simulink model "v7_2025_11_28_D2_work_in_progress"  (R2025a)
settings: Solver=FixedStepAuto  StartTime=0.0  StopTime=120  FixedStep=1e-3  RelTol=1e-3  EnableMultiTasking=on
undefined symbols (not defined in the file): A0, A1, D0, D1, D10, D11, D12, D13, D2, D3, D4, D5, D6, D7, D8, D9, PTA0, PTA1, PTA2, PTB2, PTB23, PTB3, PTB9, PTC16, PTC17, PTC2, PTC3, PTC4, PTD0, PTD1, PTD2, PTD3
libraries: frdmk64flib x19, etargetslib x2, dspstat3 x1
settings Model: ExtModeTrigDuration=5  Creator=School Account  LastModifiedBy=School Account
settings SolverCC: AlgebraicLoopSolver=TrustRegion  AutoInsertRateTranBlk=on
settings OptimizationCC: DefaultParameterBehavior=Inlined  EnhancedBackFolding=on  PassReuseOutputArgsAs=Individual arguments  ZeroExternalMemoryAtStartup=off  ZeroInternalMemoryAtStartup=off  MaxStackSize=64  OptimizeBlockOrder=speed  DifferentSizesBufferReuse=on  OptimizationCustomize=off  EfficientTunableParamExpr=on
settings DebuggingCC: ParameterTunabilityLossMsg=error
settings HardwareCC: ProdBitPerPointer=32.0  ProdBitPerSizeT=32.0  ProdBitPerPtrDiffT=32.0  ProdLargestAtomicInteger=Long  ProdLargestAtomicFloat=Double  ProdWordSize=32.0  ProdHWDeviceType=ARM Compatible->ARM Cortex
settings SFSimCC: MATLABDynamicMemAlloc=off
settings RTWCC: SystemTargetFile=ert.tlc  HardwareBoard=NXP FRDM-K64F  TLCOptions="-aInlineSetEventsForThisBaseRateFcn=TLC_FALSE -aSuppressMultiTaskScheduler=TLC_FALSE  -aRateBasedStepFcn=0"  TemplateMakefile=ert_default_tmf  Toolchain=GNU Tools for ARM Embedded Processors  GPUComputeCapability=3.5  Description=Embedded Coder
settings CodeAppCC: ForceParamTrailComments=on  IgnoreCustomStorageClasses=off  OperatorAnnotations=on  SimulinkDataObjDesc=on  SFDataObjDesc=on  InsertBlockDesc=on
settings ERTTargetCC: ExtModeTransport=4.0  ExtModeStaticAlloc=off  ExtModeMexFile=sendToCommService  ExtModeIntrfLevel=Level1  DynamicArrayContainerType=coder::array

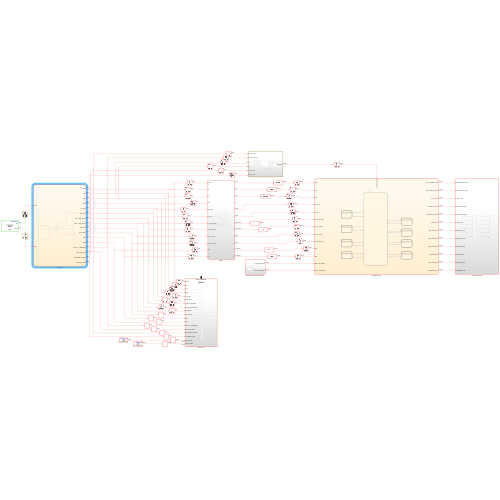
[thumbnail: Simulink's stored preview of the top-level diagram]
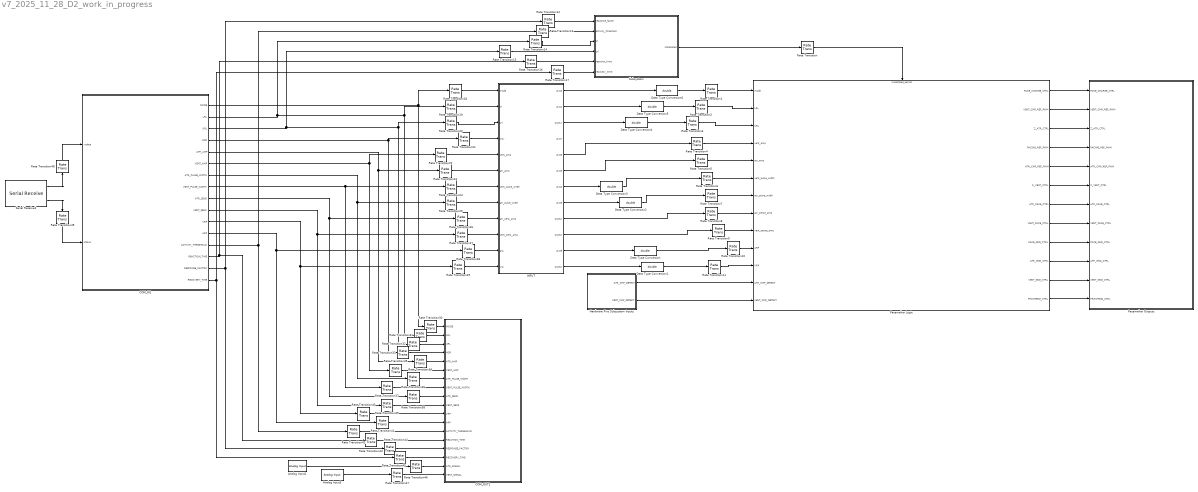
== system v7_2025_11_28_D2_work_in_progress ==
  Analog Input2 : frdmk64flib/Analog Input  Whichpin=PTB2 (A0)  SampleTime=-1
  Analog Input3 : frdmk64flib/Analog Input  Whichpin=PTB3 (A1)  SampleTime=-1
  COM_IN1 : Stateflow chart  TreatAsAtomicUnit=on
  COM_OUT1 : Subsystem  TreatAsAtomicUnit=on
  Data Type Conversion{,1..6} (7 alike) : DataTypeConversion  OutDataTypeStr=double  SaturateOnIntegerOverflow=off  RndMeth=Floor
  Hardware Pins Subsystem Inputs : Subsystem
  "INPUT " : Subsystem
  Pacemaker Logic : Stateflow chart  TreatAsAtomicUnit=on
      settings: PortSchema="{\"entries\":[{\"content\":{\"sides\":[{\"content\":{\"connectorIds\":[\"In1\",\"In4\",\"In13\",\"In5\",\"In2\",\"In6\",\"In3\",\"In7\",\"In10\",\"In8\",\"In11\",\"In9\",\"In12\"]},\"type\":\"ConnectorPlacement.EquallySpacedRectSide\",\"uuid\":\"2821f65a-9b3e-4ca7-babd-b0602bfdca31\"},{\"content\":{\"connectorIds\":[\"Out1\",\"Out2\",\"Out3\",\"Out4\",\"Out5\",\"Out6\",\"Out7\",\"Out8\",\"Out9\",\"Out10\",\"Out11\",\"Out12\"],\"side\":\"RIGHT\"},\"type\":\"ConnectorPlacement.EquallySpacedRectSide\",\"uuid\":\"3302ad84-7e85-4bae-9388-240b69681e7f\"},{\"content\":{\"connectorIds\":[\"In14\"],\"side\":\"TOP\"},\"type\":\"ConnectorPlacement.EquallySpacedRectSide\",\"uuid\":\"cc666da6-1c79-42dc-9f95-9791247ae8bf\"},{\"content\":{\"side\":\"BOTTOM\"},\"type\":\"ConnectorPlacement.EquallySpacedRectSide\",\"uuid\":\"6c7eefe5-bab4-42c2-8766-4f3cee9532f0\"}]},\"type\":\"ConnectorPlacement.EquallySpacedConnector\",\"uuid\":\"e2a43bfa-d126-4f35-adbf-2cf33da0501f\"}],\"packageUris\":[\"http://schema.mathworks.com/mf0/Connector/R2020b\"],\"version\":\"1.0\"}"
  Pacemaker Outputs : Subsystem
  Rate Transition{,1..49} (50 alike) : RateTransition  OutPortSampleTime=0.001
  Serial Receive2 : frdmk64flib/Serial Receive  SCIModule=0  Baudrate=uint32(9600)  Parity=None  StopBits=1  HardwareFlowControl=None  ByteOrder=LittleEndian  DataType=uint8  DataLength=18  BlockingMode=off  OutputStatus=on  SampleTime=0.01
  Subsystem : Subsystem
  wires:
  Pacemaker Logic/1(PACE_CHARGE_CTRL) -> Pacemaker Outputs/1(PACE_CHARGE_CTRL)
  Pacemaker Logic/3(Z_ATR_CTRL) -> Pacemaker Outputs/3(Z_ATR_CTRL)
  Pacemaker Logic/4(PACING_REF_PWM) -> Pacemaker Outputs/4(PACING_REF_PWM)
  Pacemaker Logic/7(ATR_PACE_CTRL) -> Pacemaker Outputs/7(ATR_PACE_CTRL)
  Pacemaker Logic/9(PACE_GND_CTRL) -> Pacemaker Outputs/9(PACE_GND_CTRL)
  Pacemaker Logic/10(ATR_GND_CTRL) -> Pacemaker Outputs/10(ATR_GND_CTRL)
  Pacemaker Logic/11(VENT_GND_CTRL) -> Pacemaker Outputs/11(VENT_GND_CTRL)
  Pacemaker Logic/8(VENT_PACE_CTRL) -> Pacemaker Outputs/8(VENT_PACE_CTRL)
  Pacemaker Logic/6(Z_VENT_CTRL) -> Pacemaker Outputs/6(Z_VENT_CTRL)
  Pacemaker Logic/12(FRONTEND_CTRL) -> Pacemaker Outputs/12(FRONTEND_CTRL)
  Pacemaker Logic/5(ATR_CMP_REF_PWM) -> Pacemaker Outputs/5(ATR_CMP_REF_PWM)
  Pacemaker Logic/2(VENT_CMP_REF_PWM) -> Pacemaker Outputs/2(VENT_CMP_REF_PWM)
  Hardware Pins Subsystem Inputs/2(VENT_CMP_DETECT) -> Pacemaker Logic/12(VENT_CMP_DETECT)
  Hardware Pins Subsystem Inputs/1(ATR_CMP_DETECT) -> Pacemaker Logic/9(ATR_CMP_DETECT)
  "INPUT "/11(Out9) -> Data Type Conversion/1
  "INPUT "/12(Out10) -> Data Type Conversion1/1
  "INPUT "/10(Out13) -> Rate Transition9/1
  "INPUT "/9(Out12) -> Rate Transition8/1
  "INPUT "/8(Out5) -> Data Type Conversion2/1
  "INPUT "/7(Out4) -> Data Type Conversion3/1
  "INPUT "/6(Out3) -> Rate Transition5/1
  "INPUT "/5(Out6) -> Rate Transition4/1
  "INPUT "/1(Out2) -> Data Type Conversion6/1
  "INPUT "/2(Out1) -> Data Type Conversion5/1
  "INPUT "/3(Out11) -> Data Type Conversion4/1
  Subsystem/1(Modulated) -> Rate Transition/1
  Analog Input3/1 -> Rate Transition47/1
  Analog Input2/1 -> Rate Transition46/1
  Serial Receive2/1 -> Rate Transition48/1
  Serial Receive2/2 -> Rate Transition49/1
  COM_IN1/1(MODE) -> Rate Transition18/1, Rate Transition30/1
  COM_IN1/2(LRL) -> Rate Transition14/1, Rate Transition31/1, Rate Transition19/1
  COM_IN1/3(URL) -> Rate Transition15/1, Rate Transition32/1, Rate Transition20/1
  COM_IN1/4(MSR) -> Rate Transition21/1, Rate Transition33/1
  COM_IN1/5(ATR_AMP) -> Rate Transition34/1, Rate Transition23/1
  COM_IN1/6(VENT_AMP) -> Rate Transition22/1, Rate Transition35/1
  COM_IN1/7(ATR_PULSE_WIDTH) -> Rate Transition36/1, Rate Transition25/1
  COM_IN1/8(VENT_PULSE_WIDTH) -> Rate Transition37/1, Rate Transition24/1
  COM_IN1/9(ATR_SENS) -> Rate Transition26/1, Rate Transition38/1
  COM_IN1/10(VENT_SENS) -> Rate Transition27/1, Rate Transition39/1
  COM_IN1/11(VRP) -> Rate Transition29/1, Rate Transition40/1
  COM_IN1/12(ARP) -> Rate Transition28/1, Rate Transition41/1
  COM_IN1/13(ACTIVITY_THRESHOLD) -> Rate Transition13/1, Rate Transition42/1
  COM_IN1/14(REACTION_TIME) -> Rate Transition16/1, Rate Transition43/1
  COM_IN1/15(RESPONSE_FACTOR) -> Rate Transition12/1, Rate Transition44/1
  COM_IN1/16(RECOVERY_TIME) -> Rate Transition17/1, Rate Transition45/1
  Rate Transition/1 -> Pacemaker Logic/14(modulated_period)
  Rate Transition1/1 -> Pacemaker Logic/1(mode)
  Rate Transition2/1 -> Pacemaker Logic/4(LRL)
  Rate Transition3/1 -> Pacemaker Logic/13(URL)
  Rate Transition4/1 -> Pacemaker Logic/5(vent_amp)
  Rate Transition5/1 -> Pacemaker Logic/2(atr_amp)
  Rate Transition6/1 -> Pacemaker Logic/6(vent_pulse_width)
  Rate Transition7/1 -> Pacemaker Logic/3(atr_pulse_width)
  Rate Transition8/1 -> Pacemaker Logic/7(atr_sense_amp)
  Rate Transition9/1 -> Pacemaker Logic/10(vent_sense_amp)
  Rate Transition10/1 -> Pacemaker Logic/8(ARP)
  Rate Transition11/1 -> Pacemaker Logic/11(VRP)
  Rate Transition12/1 -> Subsystem/1(response_factor)
  Rate Transition13/1 -> Subsystem/2(activity_threshold)
  Rate Transition14/1 -> Subsystem/3(lrl)
  Rate Transition15/1 -> Subsystem/4(url)
  Rate Transition16/1 -> Subsystem/5(reaction_time)
  Rate Transition17/1 -> Subsystem/6(recovery_time)
  Rate Transition18/1 -> "INPUT "/1(mode)
  Rate Transition19/1 -> "INPUT "/2(lrl)
  Rate Transition20/1 -> "INPUT "/3(url)
  Rate Transition21/1 -> "INPUT "/4(msr)
  Rate Transition22/1 -> "INPUT "/5(vent_amp)
  Rate Transition23/1 -> "INPUT "/6(atr_amp)
  Rate Transition24/1 -> "INPUT "/7(vent_pulse_width)
  Rate Transition25/1 -> "INPUT "/8(atr_pulse_width)
  Rate Transition26/1 -> "INPUT "/9(atr_sens_amp)
  Rate Transition27/1 -> "INPUT "/10(vent_sens_amp)
  Rate Transition28/1 -> "INPUT "/11(arp)
  Rate Transition29/1 -> "INPUT "/12(vrp)
  Rate Transition30/1 -> COM_OUT1/1(MODE)
  Rate Transition31/1 -> COM_OUT1/2(LRL)
  Rate Transition32/1 -> COM_OUT1/3(URL)
  Rate Transition33/1 -> COM_OUT1/4(MSR)
  Rate Transition34/1 -> COM_OUT1/5(ATR_AMP)
  Rate Transition35/1 -> COM_OUT1/6(VENT_AMP)
  Rate Transition36/1 -> COM_OUT1/7(ATR_PULSE_WIDTH)
  Rate Transition37/1 -> COM_OUT1/8(VENT_PULSE_WIDTH)
  Rate Transition38/1 -> COM_OUT1/9(ATR_SENS)
  Rate Transition39/1 -> COM_OUT1/10(VENT_SENS)
  Rate Transition40/1 -> COM_OUT1/11(VRP)
  Rate Transition41/1 -> COM_OUT1/12(ARP)
  Rate Transition42/1 -> COM_OUT1/13(ACTIVITY_THRESHOLD)
  Rate Transition43/1 -> COM_OUT1/14(REACTION_TIME)
  Rate Transition44/1 -> COM_OUT1/15(RESPONSE_FACTOR)
  Rate Transition45/1 -> COM_OUT1/16(RECOVERY_TIME)
  Rate Transition46/1 -> COM_OUT1/17(ATR_SIGNAL)
  Rate Transition47/1 -> COM_OUT1/18(VENT_SIGNAL)
  Rate Transition48/1 -> COM_IN1/1(rxdata)
  Rate Transition49/1 -> COM_IN1/2(status)
  Data Type Conversion/1 -> Rate Transition10/1
  Data Type Conversion1/1 -> Rate Transition11/1
  Data Type Conversion2/1 -> Rate Transition7/1
  Data Type Conversion3/1 -> Rate Transition6/1
  Data Type Conversion4/1 -> Rate Transition3/1
  Data Type Conversion5/1 -> Rate Transition2/1
  Data Type Conversion6/1 -> Rate Transition1/1

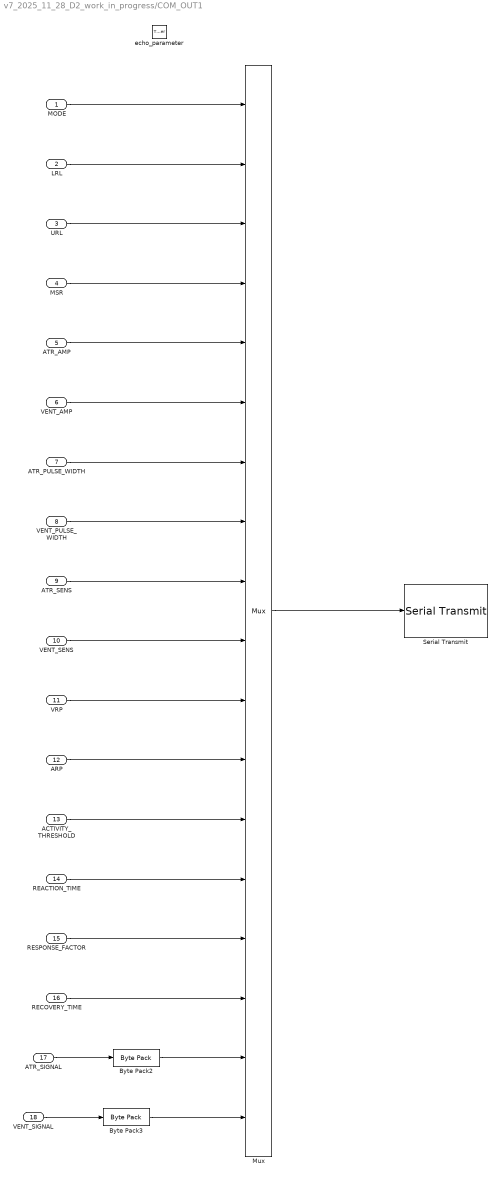
== system v7_2025_11_28_D2_work_in_progress/COM_OUT1 ==
  MODE : Inport
  LRL : Inport  Port=2
  URL : Inport  Port=3
  MSR : Inport  Port=4
  ATR_AMP : Inport  Port=5
  VENT_AMP : Inport  Port=6
  ATR_PULSE_WIDTH : Inport  Port=7
  VENT_PULSE_WIDTH : Inport  Port=8
  ATR_SENS : Inport  Port=9
  VENT_SENS : Inport  Port=10
  VRP : Inport  Port=11
  ARP : Inport  Port=12
  ACTIVITY_THRESHOLD : Inport  Port=13
  REACTION_TIME : Inport  Port=14
  RESPONSE_FACTOR : Inport  Port=15
  RECOVERY_TIME : Inport  Port=16
  ATR_SIGNAL : Inport  Port=17  OutDataTypeStr=double
  VENT_SIGNAL : Inport  Port=18  OutDataTypeStr=double
  echo_parameter : TriggerPort  TriggerType=function-call  IsSimulinkFunction=on  FunctionName=echo_parameter  VariantControl=(inherit)
  Byte Pack2 : etargetslib/Byte Pack  datatypes={'double'}  byteAlign=1
  Byte Pack3 : etargetslib/Byte Pack  datatypes={'double'}  byteAlign=1
  Mux : Mux  Inputs=18
  Serial Transmit : frdmk64flib/Serial Transmit  SCIModule=0  Baudrate=uint32(9600)  Parity=None  StopBits=1  HardwareFlowControl=None  ByteOrder=LittleEndian  BlockingMode=on  OutputStatus=off
  wires:
  VENT_SIGNAL/1 -> Byte Pack3/1
  ATR_SIGNAL/1 -> Byte Pack2/1
  Byte Pack2/1 -> Mux/17
  Byte Pack3/1 -> Mux/18
  Mux/1 -> Serial Transmit/1
  MODE/1 -> Mux/1
  LRL/1 -> Mux/2
  URL/1 -> Mux/3
  MSR/1 -> Mux/4
  ATR_AMP/1 -> Mux/5
  VENT_AMP/1 -> Mux/6
  ATR_PULSE_WIDTH/1 -> Mux/7
  VENT_PULSE_WIDTH/1 -> Mux/8
  ATR_SENS/1 -> Mux/9
  VENT_SENS/1 -> Mux/10
  VRP/1 -> Mux/11
  ARP/1 -> Mux/12
  ACTIVITY_THRESHOLD/1 -> Mux/13
  REACTION_TIME/1 -> Mux/14
  RESPONSE_FACTOR/1 -> Mux/15
  RECOVERY_TIME/1 -> Mux/16

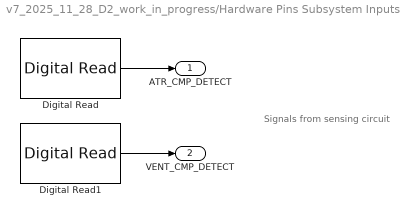
== system v7_2025_11_28_D2_work_in_progress/Hardware Pins Subsystem Inputs ==
  note: Signals from sensing circuit
  Digital Read : frdmk64flib/Digital Read  Whichpin=PTC16 (D0)  SampleTime=-1
  Digital Read1 : frdmk64flib/Digital Read  Whichpin=PTC17 (D1)  SampleTime=-1
  ATR_CMP_DETECT : Outport
  VENT_CMP_DETECT : Outport  Port=2
  wires:
  Digital Read1/1 -> VENT_CMP_DETECT/1
  Digital Read/1 -> ATR_CMP_DETECT/1

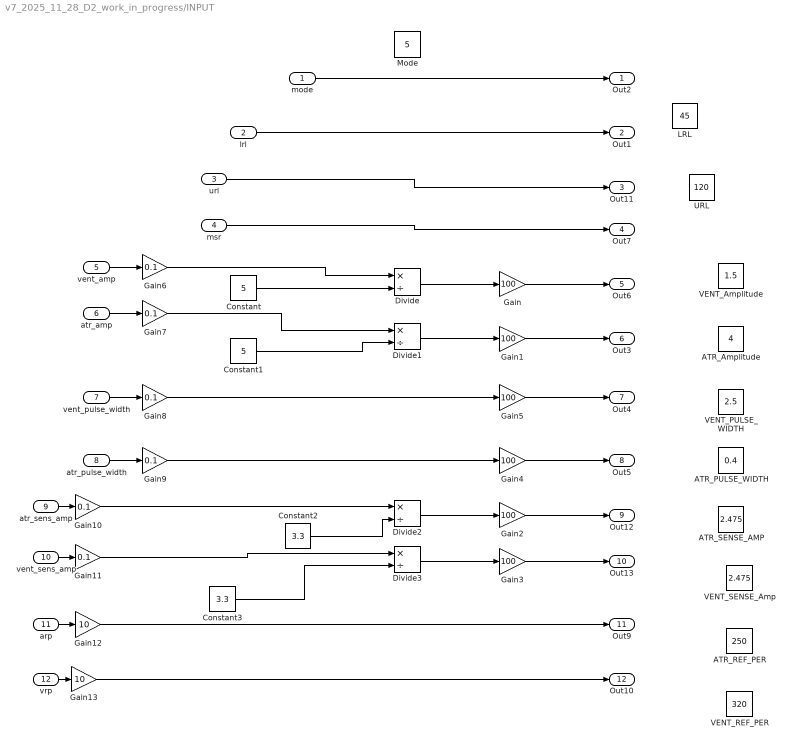
== system v7_2025_11_28_D2_work_in_progress/INPUT  ==
  mode : Inport
  lrl : Inport  Port=2
  url : Inport  Port=3
  msr : Inport  Port=4
  vent_amp : Inport  Port=5
  atr_amp : Inport  Port=6
  vent_pulse_width : Inport  Port=7
  atr_pulse_width : Inport  Port=8
  atr_sens_amp : Inport  Port=9
  vent_sens_amp : Inport  Port=10
  arp : Inport  Port=11
  vrp : Inport  Port=12
  ATR_Amplitude : Constant  Value=4
  ATR_PULSE_WIDTH : Constant  Value=0.4
  ATR_REF_PER : Constant  Value=250
  ATR_SENSE_AMP : Constant  Value=2.475
  Constant : Constant  Value=5
  Constant1 : Constant  Value=5
  Constant2 : Constant  Value=3.3
  Constant3 : Constant  Value=3.3
  Divide{,1..3} (4 alike) : Product  Inputs=*/
  Gain{,1..5} (6 alike) : Gain  Gain=100
  Gain{6..11} (6 alike) : Gain  Gain=0.1
  Gain12 : Gain  Gain=10
  Gain13 : Gain  Gain=10
  LRL : Constant  Value=45
  Mode : Constant  Value=5
  URL : Constant  Value=120
  VENT_Amplitude : Constant  Value=1.5
  VENT_PULSE_WIDTH : Constant  Value=2.5
  VENT_REF_PER : Constant  Value=320
  VENT_SENSE_Amp : Constant  Value=2.475
  Out2 : Outport
  Out1 : Outport  Port=2
  Out11 : Outport  Port=3
  Out7 : Outport  Port=4
  Out6 : Outport  Port=5
  Out3 : Outport  Port=6
  Out4 : Outport  Port=7
  Out5 : Outport  Port=8
  Out12 : Outport  Port=9
  Out13 : Outport  Port=10
  Out9 : Outport  Port=11
  Out10 : Outport  Port=12
  wires:
  Gain/1 -> Out6/1
  Gain1/1 -> Out3/1
  Gain2/1 -> Out12/1
  Gain3/1 -> Out13/1
  Gain5/1 -> Out4/1
  Gain4/1 -> Out5/1
  Divide/1 -> Gain/1
  Constant/1 -> Divide/2
  Divide1/1 -> Gain1/1
  Constant1/1 -> Divide1/2
  Divide2/1 -> Gain2/1
  Constant2/1 -> Divide2/2
  Divide3/1 -> Gain3/1
  Constant3/1 -> Divide3/2
  vent_amp/1 -> Gain6/1
  mode/1 -> Out2/1
  lrl/1 -> Out1/1
  url/1 -> Out11/1
  msr/1 -> Out7/1
  atr_amp/1 -> Gain7/1
  vent_pulse_width/1 -> Gain8/1
  Gain8/1 -> Gain5/1
  atr_pulse_width/1 -> Gain9/1
  Gain9/1 -> Gain4/1
  atr_sens_amp/1 -> Gain10/1
  Gain6/1 -> Divide/1
  Gain7/1 -> Divide1/1
  Gain10/1 -> Divide2/1
  vent_sens_amp/1 -> Gain11/1
  Gain11/1 -> Divide3/1
  arp/1 -> Gain12/1
  vrp/1 -> Gain13/1
  Gain12/1 -> Out9/1
  Gain13/1 -> Out10/1

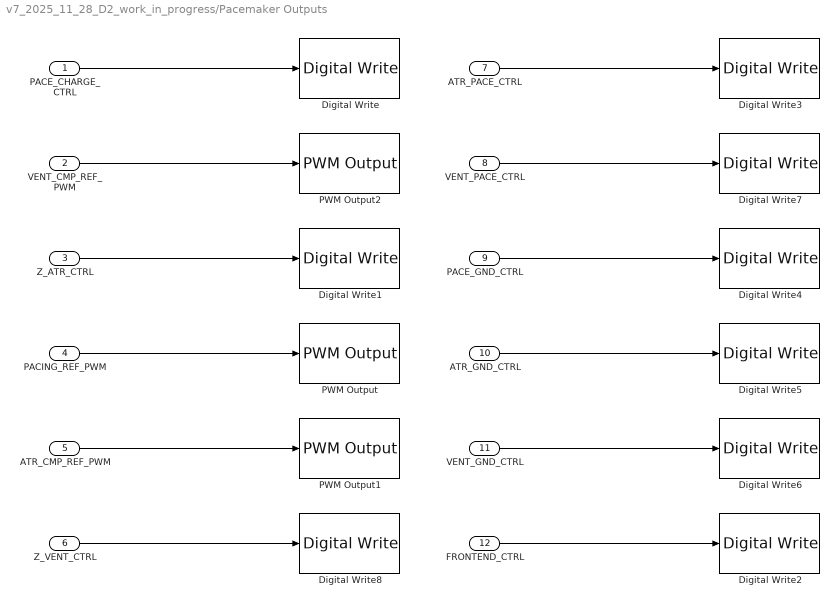
== system v7_2025_11_28_D2_work_in_progress/Pacemaker Outputs ==
  PACE_CHARGE_CTRL : Inport
  VENT_CMP_REF_PWM : Inport  Port=2
  Z_ATR_CTRL : Inport  Port=3
  PACING_REF_PWM : Inport  Port=4
  ATR_CMP_REF_PWM : Inport  Port=5
  Z_VENT_CTRL : Inport  Port=6
  ATR_PACE_CTRL : Inport  Port=7
  VENT_PACE_CTRL : Inport  Port=8
  PACE_GND_CTRL : Inport  Port=9
  ATR_GND_CTRL : Inport  Port=10
  VENT_GND_CTRL : Inport  Port=11
  FRONTEND_CTRL : Inport  Port=12
  Digital Write : frdmk64flib/Digital Write  Whichpin=PTB9 (D2)
  Digital Write1 : frdmk64flib/Digital Write  Whichpin=PTB23 (D4)
  Digital Write2 : frdmk64flib/Digital Write  Whichpin=PTD1 (D13)
  Digital Write3 : frdmk64flib/Digital Write  Whichpin=PTA0 (D8)
  Digital Write4 : frdmk64flib/Digital Write  Whichpin=PTD0 (D10)
  Digital Write5 : frdmk64flib/Digital Write  Whichpin=PTD2 (D11)
  Digital Write6 : frdmk64flib/Digital Write  Whichpin=PTD3 (D12)
  Digital Write7 : frdmk64flib/Digital Write  Whichpin=PTC4 (D9)
  Digital Write8 : frdmk64flib/Digital Write  Whichpin=PTC3 (D7)
  PWM Output : frdmk64flib/PWM Output  Whichpin=PTA2 (D5)  InitialFrequency=2000  InitialDutyCycle=0
  PWM Output1 : frdmk64flib/PWM Output  Whichpin=PTC2 (D6)  InitialFrequency=2000  InitialDutyCycle=0
  PWM Output2 : frdmk64flib/PWM Output  Whichpin=PTA1 (D3)  InitialFrequency=2000  InitialDutyCycle=0
  wires:
  PACE_CHARGE_CTRL/1 -> Digital Write/1
  Z_ATR_CTRL/1 -> Digital Write1/1
  PACING_REF_PWM/1 -> PWM Output/1
  ATR_PACE_CTRL/1 -> Digital Write3/1
  PACE_GND_CTRL/1 -> Digital Write4/1
  ATR_GND_CTRL/1 -> Digital Write5/1
  VENT_GND_CTRL/1 -> Digital Write6/1
  VENT_PACE_CTRL/1 -> Digital Write7/1
  Z_VENT_CTRL/1 -> Digital Write8/1
  FRONTEND_CTRL/1 -> Digital Write2/1
  ATR_CMP_REF_PWM/1 -> PWM Output1/1
  VENT_CMP_REF_PWM/1 -> PWM Output2/1

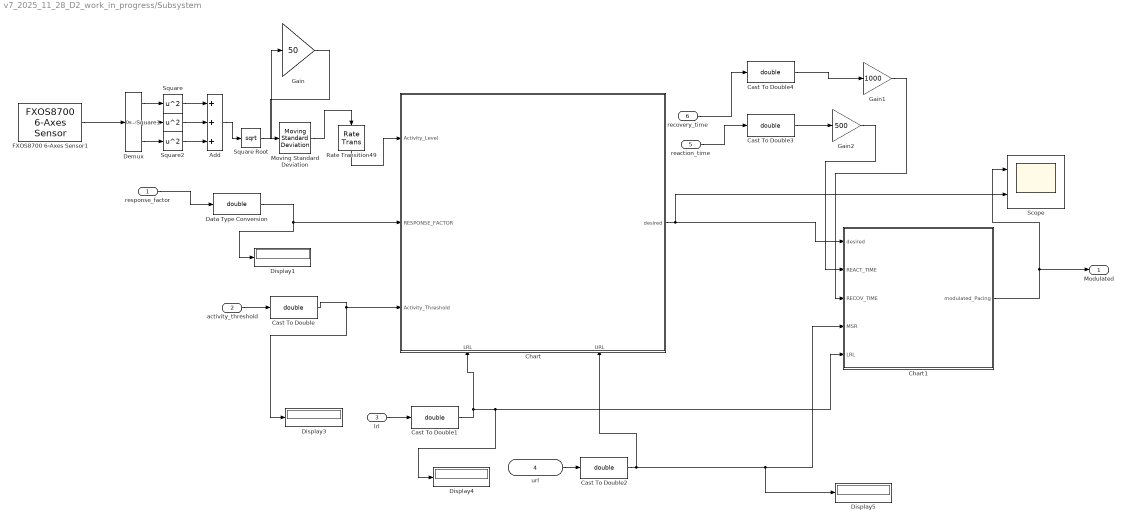
== system v7_2025_11_28_D2_work_in_progress/Subsystem ==
  response_factor : Inport
  activity_threshold : Inport  Port=2
  lrl : Inport  Port=3
  url : Inport  Port=4
  reaction_time : Inport  Port=5
  recovery_time : Inport  Port=6
  Add : Sum  Inputs=+++
  Cast To Double{,1..4} (5 alike) : DataTypeConversion  OutDataTypeStr=double  SaturateOnIntegerOverflow=off  RndMeth=Floor
  Chart : Stateflow chart  TreatAsAtomicUnit=on
      settings: PortSchema="{\"entries\":[{\"content\":{\"sides\":[{\"content\":{\"connectorIds\":[\"In3\",\"In4\",\"In5\"]},\"type\":\"ConnectorPlacement.EquallySpacedRectSide\",\"uuid\":\"74c786d3-d2a6-437e-8bb7-c9d9b4a74617\"},{\"content\":{\"connectorIds\":[\"Out1\"],\"side\":\"RIGHT\"},\"type\":\"ConnectorPlacement.EquallySpacedRectSide\",\"uuid\":\"2c46704d-1ce5-4a26-9635-57e0f6503ead\"},{\"content\":{\"side\":\"TOP\"},\"type\":\"ConnectorPlacement.EquallySpacedRectSide\",\"uuid\":\"1e7c0bb1-a8b6-49e0-9e63-e8e48adc5546\"},{\"content\":{\"connectorIds\":[\"In1\",\"In2\"],\"side\":\"BOTTOM\"},\"type\":\"ConnectorPlacement.EquallySpacedRectSide\",\"uuid\":\"98fe2a4d-8dd5-42bc-97d4-b5234350e537\"}]},\"type\":\"ConnectorPlacement.EquallySpacedConnector\",\"uuid\":\"114a6ead-843c-4291-bcbc-4dc58f15d580\"}],\"packageUris\":[\"http://schema.mathworks.com/mf0/Connector/R2020b\"],\"version\":\"1.0\"}"
  Chart1 : Stateflow chart  TreatAsAtomicUnit=on
  Data Type Conversion : DataTypeConversion  OutDataTypeStr=double  SaturateOnIntegerOverflow=off  RndMeth=Floor
  Demux : Demux  Outputs=3
  Display{1,3..5} (4 alike) : Display
  FXOS8700 6-Axes Sensor1 : frdmk64flib/FXOS8700 6-Axes Sensor  Activesensor=Accelerometer only  ODR=800Hz  HybridODR=400Hz  Accelfullrange=-4g to +4g  SampleTime=0.01
  Gain : Gain  Gain=50
  Gain1 : Gain  Gain=1000
  Gain2 : Gain  Gain=500
  Moving Standard Deviation : dspstat3/Moving Standard Deviation  Method=Sliding window  ForgettingFactorPort=off  SpecifyWindowLength=on  WindowLength=128  OverlapLength=127  AllowArbitraryInputLength=off  ForgettingFactor=0.9  SimulateUsing=Interpreted execution
  Rate Transition49 : RateTransition  OutPortSampleTime=0.001
  Scope : Scope  NumInputPorts=2
      settings: ActiveDisplayYMinimum=34.87115106781259  ActiveDisplayYMaximum=115.78130537109008
  Square : Math  Operator=square
  Square Root : Sqrt
  Square1 : Math  Operator=square
  Square2 : Math  Operator=square
  Modulated : Outport
  wires:
  Square1/1 -> Add/2
  Demux/1 -> Square/1
  Square2/1 -> Add/3
  Square/1 -> Add/1
  Demux/2 -> Square1/1
  Demux/3 -> Square2/1
  Add/1 -> Square Root/1
  FXOS8700 6-Axes Sensor1/1 -> Demux/1
  Chart1/1(modulated_Pacing) -> Modulated/1, Scope/1
  Chart/1(desired) -> Chart1/1(desired), Scope/2
  Square Root/1 -> Gain/1
  Gain/1 -> Moving Standard Deviation/1
  response_factor/1 -> Data Type Conversion/1
  Data Type Conversion/1 -> Display1/1, Chart/4(RESPONSE_FACTOR)
  activity_threshold/1 -> Cast To Double/1
  lrl/1 -> Cast To Double1/1
  url/1 -> Cast To Double2/1
  Cast To Double1/1 -> Display4/1, Chart1/5(LRL), Chart/1(LRL)
  Cast To Double2/1 -> Chart/2(URL), Display5/1, Chart1/4(MSR)
  recovery_time/1 -> Cast To Double4/1
  reaction_time/1 -> Cast To Double3/1
  Cast To Double4/1 -> Gain1/1
  Cast To Double/1 -> Chart/5(Activity_Threshold), Display3/1
  Gain1/1 -> Chart1/3(RECOV_TIME)
  Cast To Double3/1 -> Gain2/1
  Gain2/1 -> Chart1/2(REACT_TIME)
  Moving Standard Deviation/1 -> Rate Transition49/1
  Rate Transition49/1 -> Chart/3(Activity_Level)

== stateflow chart v7_2025_11_28_D2_work_in_progress/Subsystem/Chart ==
  state UpperLimiter [commented out]
    entry:
    desired = URL
  state LinearFunction
    during:
    desired = RESPONSE_FACTOR * (Activity_Level  -  Activity_Threshold) + LRL
    % 2. Apply Upper Limit (Clamp to URL)
    if desired > URL
    desired = URL;
    % 3. Apply Lower Limit (Clamp to LRL)
    elseif desired < LRL
    desired = LRL;
    end
  state Init
    entry:
    desired = LRL
  state Start
  state LowerLimiter [commented out]
    entry:
    desired = LRL
  LinearFunction -> UpperLimiter [commented out] : [desired > URL]
  UpperLimiter -> LinearFunction [commented out] : [desired <= URL]
  (default) -> Init
  Init -> Start
  Start -> LinearFunction : [Activity_Level >= Activity_Threshold]
  LinearFunction -> Start : [Activity_Level < Activity_Threshold]
  LowerLimiter -> LinearFunction [commented out] : [desired >= LRL]
  LinearFunction -> LowerLimiter [commented out] : [desired < LRL]
  data: LRL input; URL input; Activity_Level input; RESPONSE_FACTOR input; Activity_Threshold input; desired output

== stateflow chart v7_2025_11_28_D2_work_in_progress/Subsystem/Chart1 ==
  state Pacing_Up [commented out]
    during:
    % --- SLOW MODE ---
    % Multiply by 2 (or more) to extend the time.
    % Example: 5 seconds becomes 10 seconds.
    local_react = double(REACT_TIME) * 2;
    % Safety: Prevent divide by zero if input is missing
    if local_react < 100
    local_react = 1000; % Default to 1 second
    end
    % --- CALCULATION ---
    % Calculate step size.
    % Note: Using (MSR-LRL) creates a steady straight line.
    % Using (desired-modulated) creates a curved line.
    increment = (double(MSR) - double(LRL)) / local_react;
    % Apply
    modulated_Pacing = modulated_Pacing + increment;
    % Clamp
    if modulated_Pacing > MSR
    modulated_Pacing = double(MSR);
    end
  state Steady_State_ [commented out]
    during:
    difference = desired - modulated_Pacing;
  state Init1 [commented out]
    entry:
    modulated_Pacing=double(LRL);
  state Pacing_Up1
    during:
    % Calculate the step size needed to close the gap based on REACT_TIME
    % Doing this every step creates a smooth approach
    increment = (desired - modulated_Pacing) / REACT_TIME;
    % Apply the increment (assuming 1ms step)
    modulated_Pacing = modulated_Pacing + increment;
    % Safety Clamp: Don't go over MSR
    if modulated_Pacing > MSR
    modulated_Pacing = MSR;
    end
  state Pacing_Down [commented out]
    during:
    % --- SLOW MODE ---
    % Multiply by 5 to make it really gentle
    local_recov = double(RECOV_TIME) * 5;
    % Safety
    if local_recov < 100
    local_recov = 1000;
    end
    % --- CALCULATION ---
    % Note: LRL - MSR gives the negative number we need
    decrement = (double(LRL) - double(MSR)) / local_recov;
    % Apply
    modulated_Pacing = modulated_Pacing + decrement;
    % Clamp
    if modulated_Pacing < LRL
    modulated_Pacing = double(LRL);
    end
  state Steady_State
    during:
    difference=desired - modulated_Pacing
  state Init2
    entry:
    modulated_Pacing=LRL
  state Pacing_Down1
    during:
    % Calculate the decrement based on RECOV_TIME
    decrement = (desired - modulated_Pacing) / RECOV_TIME;
    % Note: decrement will be negative because (desired - modulated) is negative
    % Apply the decrement
    modulated_Pacing = modulated_Pacing + decrement;
    % Safety Clamp: Don't go under LRL
    if modulated_Pacing < LRL
    modulated_Pacing = LRL;
    end
  Steady_State_ -> Pacing_Up [commented out] : [desired > modulated_Pacing]
  Pacing_Up -> Steady_State_ [commented out] : [modulated_Pacing >= desired]
  (default) -> Init1 [commented out]
  Init1 -> Steady_State_ [commented out]
  Pacing_Down -> Steady_State_ [commented out] : [modulated_Pacing <= desired]
  Steady_State_ -> Pacing_Down [commented out] : [desired < modulated_Pacing]
  Steady_State -> Pacing_Up1 [order 1] : [desired > modulated_Pacing]
  (default) -> Init2
  Pacing_Up1 -> Steady_State : [modulated_Pacing >= desired]
  Init2 -> Steady_State
  Steady_State -> Pacing_Down1 [order 2] : [desired < modulated_Pacing]
  Pacing_Down1 -> Steady_State : [modulated_Pacing <= desired]
  data: desired input; REACT_TIME input; RECOV_TIME input; modulated_Pacing output =60; difference local; increment local; decrement local; MSR input; LRL input; local_react local; local_recov local; safe_react local; safe_recov local; raw_react local; raw_recov local; SCALER local

== stateflow chart v7_2025_11_28_D2_work_in_progress/Pacemaker Logic ==
  settings: updateMethod=DISCRETE  sampleTime=0.001
  state Start
  state VVIR
    state VVI_Charge
      entry:
      FRONTEND_CTRL = 1;
      %Charging C22
      VENT_PACE_CTRL = 0;
      ATR_PACE_CTRL = 0;
      PACING_REF_PWM = vent_amp;
      PACE_CHARGE_CTRL = 1;
      %Discharging C21
      PACE_GND_CTRL = 1;
      VENT_PACE_CTRL = 0;
      Z_ATR_CTRL = 0;
      Z_VENT_CTRL = 0;
      ATR_PACE_CTRL = 0;
      ATR_GND_CTRL = 0;
      VENT_GND_CTRL = 1;
      VENT_CMP_REF_PWM = vent_sense_amp;
    state VVI_Pace
      entry:
      %Pacing
      PACE_CHARGE_CTRL = 0;
      PACE_GND_CTRL= 1;
      ATR_PACE_CTRL = 0;
      ATR_GND_CTRL= 0;
      Z_ATR_CTRL = 0;
      Z_VENT_CTRL = 0;
      VENT_GND_CTRL = 0;
      VENT_PACE_CTRL = 1;
    state VVI_Inhibit
      entry:
      FRONTEND_CTRL = 0;
      %Charging C22
      VENT_PACE_CTRL = 0;
      ATR_PACE_CTRL = 0;
      PACING_REF_PWM = vent_amp;
      PACE_CHARGE_CTRL = 1;
      %Discharging C21
      PACE_GND_CTRL = 1;
      VENT_PACE_CTRL = 0;
      Z_VENT_CTRL = 0;
      Z_ATR_CTRL = 0;
      ATR_PACE_CTRL = 0;
      ATR_GND_CTRL = 0;
      VENT_GND_CTRL = 1;
      VENT_CMP_REF_PWM = vent_sense_amp;
    (default) -> VVIR.VVI_Charge
    VVIR.VVI_Charge -> VVIR.VVI_Pace [order 1] : [after(60000/modulated_period - vent_pulse_width - VRP,msec)]
    VVIR.VVI_Charge -> (junction 112) [order 2] : [VENT_CMP_DETECT == 1]
    (junction 112) -> VVIR.VVI_Inhibit : [after(vent_pulse_width,msec)]
    VVIR.VVI_Pace -> VVIR.VVI_Inhibit : [after(vent_pulse_width,msec)]
    VVIR.VVI_Inhibit -> VVIR.VVI_Charge : [after(VRP, msec)]
  state VVI
    state VVI_Charge
      entry:
      FRONTEND_CTRL = 1;
      %Charging C22
      VENT_PACE_CTRL = 0;
      ATR_PACE_CTRL = 0;
      PACING_REF_PWM = vent_amp;
      PACE_CHARGE_CTRL = 1;
      %Discharging C21
      PACE_GND_CTRL = 1;
      VENT_PACE_CTRL = 0;
      Z_ATR_CTRL = 0;
      Z_VENT_CTRL = 0;
      ATR_PACE_CTRL = 0;
      ATR_GND_CTRL = 0;
      VENT_GND_CTRL = 1;
      VENT_CMP_REF_PWM = vent_sense_amp;
    state VVI_Pace
      entry:
      %Pacing
      PACE_CHARGE_CTRL = 0;
      PACE_GND_CTRL= 1;
      ATR_PACE_CTRL = 0;
      ATR_GND_CTRL= 0;
      Z_ATR_CTRL = 0;
      Z_VENT_CTRL = 0;
      VENT_GND_CTRL = 0;
      VENT_PACE_CTRL = 1;
    state VVI_Inhibit
      entry:
      FRONTEND_CTRL = 0;
      %Charging C22
      VENT_PACE_CTRL = 0;
      ATR_PACE_CTRL = 0;
      PACING_REF_PWM = vent_amp;
      PACE_CHARGE_CTRL = 1;
      %Discharging C21
      PACE_GND_CTRL = 1;
      VENT_PACE_CTRL = 0;
      Z_VENT_CTRL = 0;
      Z_ATR_CTRL = 0;
      ATR_PACE_CTRL = 0;
      ATR_GND_CTRL = 0;
      VENT_GND_CTRL = 1;
      VENT_CMP_REF_PWM = vent_sense_amp;
    (default) -> VVI.VVI_Charge
    VVI.VVI_Charge -> VVI.VVI_Pace [order 1] : [after(60000/LRL - vent_pulse_width - VRP,msec)]
    VVI.VVI_Charge -> (junction 65) [order 2] : [VENT_CMP_DETECT == 1]
    (junction 65) -> VVI.VVI_Inhibit : [after(vent_pulse_width,msec)]
    VVI.VVI_Pace -> VVI.VVI_Inhibit : [after(vent_pulse_width,msec)]
    VVI.VVI_Inhibit -> VVI.VVI_Charge : [after(VRP, msec)]
  state AAIR
    state AAI_Charge
      entry:
      FRONTEND_CTRL = 1;
      %Charging C22
      ATR_PACE_CTRL = 0;
      VENT_PACE_CTRL = 0;
      PACING_REF_PWM = atr_amp;
      PACE_CHARGE_CTRL = 1;
      %Discharging C21
      PACE_GND_CTRL = 1;
      ATR_PACE_CTRL = 0;
      Z_VENT_CTRL = 0;
      Z_ATR_CTRL = 0;
      VENT_PACE_CTRL = 0;
      VENT_GND_CTRL = 0;
      ATR_GND_CTRL = 1;
      ATR_CMP_REF_PWM = atr_sense_amp;
    state AAI_Pace
      entry:
      %Pacing
      PACE_CHARGE_CTRL = 0;
      PACE_GND_CTRL= 1;
      VENT_PACE_CTRL = 0;
      VENT_GND_CTRL= 0;
      Z_VENT_CTRL = 0;
      Z_ATR_CTRL = 0;
      ATR_GND_CTRL = 0;
      ATR_PACE_CTRL = 1;
    state AAI_Inhibit
      entry:
      FRONTEND_CTRL = 0;
      %Charging C22
      ATR_PACE_CTRL = 0;
      VENT_PACE_CTRL = 0;
      PACING_REF_PWM = atr_amp;
      PACE_CHARGE_CTRL = 1;
      %Discharging C21
      PACE_GND_CTRL = 1;
      ATR_PACE_CTRL = 0;
      Z_VENT_CTRL = 0;
      Z_ATR_CTRL = 0;
      VENT_PACE_CTRL = 0;
      VENT_GND_CTRL = 0;
      ATR_GND_CTRL = 1;
      ATR_CMP_REF_PWM = atr_sense_amp;
    (default) -> AAIR.AAI_Charge
    AAIR.AAI_Charge -> AAIR.AAI_Pace [order 1] : [after(60000/modulated_period - atr_pulse_width - ARP,msec)]
    AAIR.AAI_Charge -> (junction 101) [order 2] : [ATR_CMP_DETECT == 1]
    (junction 101) -> AAIR.AAI_Inhibit : [after(atr_pulse_width,msec)]
    AAIR.AAI_Pace -> AAIR.AAI_Inhibit : [after(atr_pulse_width,msec)]
    AAIR.AAI_Inhibit -> AAIR.AAI_Charge : [after(ARP, msec)]
  state AAI
    state AAI_Charge
      entry:
      FRONTEND_CTRL = 1;
      %Charging C22
      ATR_PACE_CTRL = 0;
      VENT_PACE_CTRL = 0;
      PACING_REF_PWM = atr_amp;
      PACE_CHARGE_CTRL = 1;
      %Discharging C21
      PACE_GND_CTRL = 1;
      ATR_PACE_CTRL = 0;
      Z_VENT_CTRL = 0;
      Z_ATR_CTRL = 0;
      VENT_PACE_CTRL = 0;
      VENT_GND_CTRL = 0;
      ATR_GND_CTRL = 1;
      ATR_CMP_REF_PWM = atr_sense_amp;
    state AAI_Pace
      entry:
      %Pacing
      PACE_CHARGE_CTRL = 0;
      PACE_GND_CTRL= 1;
      VENT_PACE_CTRL = 0;
      VENT_GND_CTRL= 0;
      Z_VENT_CTRL = 0;
      Z_ATR_CTRL = 0;
      ATR_GND_CTRL = 0;
      ATR_PACE_CTRL = 1;
    state AAI_Inhibit
      entry:
      FRONTEND_CTRL = 0;
      %Charging C22
      ATR_PACE_CTRL = 0;
      VENT_PACE_CTRL = 0;
      PACING_REF_PWM = atr_amp;
      PACE_CHARGE_CTRL = 1;
      %Discharging C21
      PACE_GND_CTRL = 1;
      ATR_PACE_CTRL = 0;
      Z_VENT_CTRL = 0;
      Z_ATR_CTRL = 0;
      VENT_PACE_CTRL = 0;
      VENT_GND_CTRL = 0;
      ATR_GND_CTRL = 1;
      ATR_CMP_REF_PWM = atr_sense_amp;
    (default) -> AAI.AAI_Charge
    AAI.AAI_Charge -> AAI.AAI_Pace [order 1] : [after(60000/LRL - atr_pulse_width - ARP,msec)]
    AAI.AAI_Charge -> (junction 58) [order 2] : [ATR_CMP_DETECT == 1]
    (junction 58) -> AAI.AAI_Inhibit : [after(atr_pulse_width,msec)]
    AAI.AAI_Pace -> AAI.AAI_Inhibit : [after(atr_pulse_width,msec)]
    AAI.AAI_Inhibit -> AAI.AAI_Charge : [after(ARP, msec)]
  state VOOR
    state VOO_Charge
      entry:
      FRONTEND_CTRL = 1;
      %Charging C22
      VENT_PACE_CTRL = 0;
      ATR_PACE_CTRL = 0;
      PACING_REF_PWM = vent_amp;
      PACE_CHARGE_CTRL = 1;
      %Discharging C21
      PACE_GND_CTRL = 1;
      VENT_PACE_CTRL = 0;
      Z_ATR_CTRL = 0;
      Z_VENT_CTRL = 0;
      ATR_PACE_CTRL = 0;
      ATR_GND_CTRL = 0;
      VENT_GND_CTRL = 1;
    state AOO_Pace
      entry:
      FRONTEND_CTRL = 1;
      %Pacing
      PACE_CHARGE_CTRL = 0;
      PACE_GND_CTRL= 1;
      ATR_PACE_CTRL = 0;
      ATR_GND_CTRL= 0;
      Z_ATR_CTRL = 0;
      Z_VENT_CTRL = 0;
      VENT_GND_CTRL = 0;
      VENT_PACE_CTRL = 1;
    (default) -> VOOR.VOO_Charge
    VOOR.VOO_Charge -> VOOR.AOO_Pace : [after(60000/modulated_period - vent_pulse_width,msec)]
    VOOR.AOO_Pace -> VOOR.VOO_Charge : [after(vent_pulse_width,msec)]
  state VOO
    state VOO_Charge
      entry:
      FRONTEND_CTRL = 1;
      %Charging C22
      VENT_PACE_CTRL = 0;
      ATR_PACE_CTRL = 0;
      PACING_REF_PWM = vent_amp;
      PACE_CHARGE_CTRL = 1;
      %Discharging C21
      PACE_GND_CTRL = 1;
      VENT_PACE_CTRL = 0;
      Z_ATR_CTRL = 0;
      Z_VENT_CTRL = 0;
      ATR_PACE_CTRL = 0;
      ATR_GND_CTRL = 0;
      VENT_GND_CTRL = 1;
    state AOO_Pace
      entry:
      FRONTEND_CTRL = 1;
      %Pacing
      PACE_CHARGE_CTRL = 0;
      PACE_GND_CTRL= 1;
      ATR_PACE_CTRL = 0;
      ATR_GND_CTRL= 0;
      Z_ATR_CTRL = 0;
      Z_VENT_CTRL = 0;
      VENT_GND_CTRL = 0;
      VENT_PACE_CTRL = 1;
    (default) -> VOO.VOO_Charge
    VOO.VOO_Charge -> VOO.AOO_Pace : [after(60000/LRL - vent_pulse_width,msec)]
    VOO.AOO_Pace -> VOO.VOO_Charge : [after(vent_pulse_width,msec)]
  state AOOR
    state AOO_Charge
      entry:
      FRONTEND_CTRL = 1;
      %Charging C22
      ATR_PACE_CTRL = 0;
      VENT_PACE_CTRL = 0;
      PACING_REF_PWM = atr_amp;
      PACE_CHARGE_CTRL = 1;
      %Discharging C21
      PACE_GND_CTRL = 1;
      ATR_PACE_CTRL = 0;
      Z_VENT_CTRL = 0;
      Z_ATR_CTRL = 0;
      VENT_PACE_CTRL = 0;
      VENT_GND_CTRL = 0;
      ATR_GND_CTRL = 1;
    state AOO_Pace
      entry:
      FRONTEND_CTRL = 1;
      %Pacing
      PACE_CHARGE_CTRL = 0;
      PACE_GND_CTRL= 1;
      VENT_PACE_CTRL = 0;
      VENT_GND_CTRL= 0;
      Z_VENT_CTRL = 0;
      Z_ATR_CTRL = 0;
      ATR_GND_CTRL = 0;
      ATR_PACE_CTRL = 1;
    (default) -> AOOR.AOO_Charge
    AOOR.AOO_Charge -> AOOR.AOO_Pace : [after(60000/modulated_period - atr_pulse_width,msec)]
    AOOR.AOO_Pace -> AOOR.AOO_Charge : [after(atr_pulse_width,msec)]
  state AOO
    state AOO_Charge
      entry:
      FRONTEND_CTRL = 1;
      %Charging C22
      ATR_PACE_CTRL = 0;
      VENT_PACE_CTRL = 0;
      PACING_REF_PWM = atr_amp;
      PACE_CHARGE_CTRL = 1;
      %Discharging C21
      PACE_GND_CTRL = 1;
      ATR_PACE_CTRL = 0;
      Z_VENT_CTRL = 0;
      Z_ATR_CTRL = 0;
      VENT_PACE_CTRL = 0;
      VENT_GND_CTRL = 0;
      ATR_GND_CTRL = 1;
    state AOO_Pace
      entry:
      FRONTEND_CTRL = 1;
      %Pacing
      PACE_CHARGE_CTRL = 0;
      PACE_GND_CTRL= 1;
      VENT_PACE_CTRL = 0;
      VENT_GND_CTRL= 0;
      Z_VENT_CTRL = 0;
      Z_ATR_CTRL = 0;
      ATR_GND_CTRL = 0;
      ATR_PACE_CTRL = 1;
    (default) -> AOO.AOO_Charge
    AOO.AOO_Charge -> AOO.AOO_Pace : [after(60000/LRL - atr_pulse_width,msec)]
    AOO.AOO_Pace -> AOO.AOO_Charge : [after(atr_pulse_width,msec)]
  (default) -> Start
  Start -> VVIR [order 8] : [mode == 8]
  VVIR -> Start : [mode ~= 8]
  Start -> VVI [order 6] : [mode == 4]
  VVI -> Start : [mode ~= 4]
  Start -> AAIR [order 7] : [mode == 7]
  AAIR -> Start : [mode ~= 7]
  Start -> AAI [order 5] : [mode == 3]
  AAI -> Start : [mode ~= 3]
  Start -> VOOR [order 4] : [mode == 6]
  Start -> VOO [order 1] : [mode == 2]
  VOO -> Start : [mode ~= 2]
  VOOR -> Start : [mode ~= 6]
  AOOR -> Start : [mode ~= 5]
  AOO -> Start : [mode ~= 1]
  Start -> AOO [order 2] : [mode == 1]
  Start -> AOOR [order 3] : [mode == 5]
  data: PACE_CHARGE_CTRL output; VENT_CMP_REF_PWM output; Z_ATR_CTRL output; PACING_REF_PWM output; ATR_CMP_REF_PWM output; Z_VENT_CTRL output; mode input; ATR_PACE_CTRL output; VENT_PACE_CTRL output; PACE_GND_CTRL output; atr_amp input; ATR_GND_CTRL output; atr_pulse_width input; LRL input; vent_amp input; VENT_GND_CTRL output; vent_pulse_width input; FRONTEND_CTRL output; atr_sense_amp input; ARP input; ATR_CMP_DETECT input; vent_sense_amp input; VRP input; VENT_CMP_DETECT input; URL input; modulated_period input

== stateflow chart v7_2025_11_28_D2_work_in_progress/COM_IN1 ==
  settings: executeAtInitialization=1
  state SET_PARAM
    entry:
    MODE = rxdata(3);
    LRL = rxdata(4);
    URL = rxdata(5);
    MSR = rxdata(6);
    ATR_AMP =rxdata(7);
    VENT_AMP = rxdata(8);
    ATR_PULSE_WIDTH = rxdata(9);
    VENT_PULSE_WIDTH = rxdata(10);
    ATR_SENS = rxdata(11);
    VENT_SENS = rxdata(12);
    VRP = rxdata(13);
    ARP = rxdata(14);
    ACTIVITY_THRESHOLD = rxdata(15);
    REACTION_TIME = rxdata(16);
    RESPONSE_FACTOR = rxdata(17);
    RECOVERY_TIME = rxdata(18);
  state INITIAL
    % Set the initial values of parameters
    entry:
    MODE = 3;
    LRL = 60; %60000/>LRL
    URL = 120;
    MSR = 120;
    ATR_AMP = 35; %Divide by 10
    VENT_AMP = 35; %Divide by 10
    ATR_PULSE_WIDTH = 4; %Divide by 10
    VENT_PULSE_WIDTH = 4; %Divide by 10
    ATR_SENS = 25; %Divide by 10
    VENT_SENS = 25; %Divide by 10
    VRP = 32; %Multiply by 10
    ARP = 25; %Multiply by 10
    ACTIVITY_THRESHOLD = 1;
    REACTION_TIME = 1; %Seconds
    RESPONSE_FACTOR = 1;
    RECOVERY_TIME = 1; %Minutes
  state STANDBY
    %Waiting for COM
  state ECHO_PARAM
    entry:
    echo_parameter();
  SET_PARAM -> STANDBY
  (default) -> INITIAL
  (junction 14) -> SET_PARAM [order 1] : [rxdata(2) == hex2dec('55')]
  (junction 12) -> STANDBY [order 2]
  INITIAL -> STANDBY
  STANDBY -> (junction 12) : [status == 0]
  (junction 12) -> (junction 14) [order 1] : [rxdata(1) == hex2dec('16')]
  (junction 14) -> ECHO_PARAM [order 2] : [rxdata(2) == hex2dec('22')]
  ECHO_PARAM -> STANDBY
  data: MODE output uint8; LRL output uint8; URL output uint8; MSR output uint8; rxdata input; status input; ATR_AMP output uint8; VENT_AMP output uint8; ATR_PULSE_WIDTH output uint8; VENT_PULSE_WIDTH output uint8; ATR_SENS output uint8; VENT_SENS output uint8; VRP output uint8 size=1; ARP output uint8 size=1; ACTIVITY_THRESHOLD output uint8; REACTION_TIME output uint8; RESPONSE_FACTOR output uint8; RECOVERY_TIME output uint8
